simulink model "tb_sim_monitors"  (R2026b)
undefined symbols (not defined in the file or in its folder): Ts
settings Model: Creator=aomar  LastModifiedBy=aomar

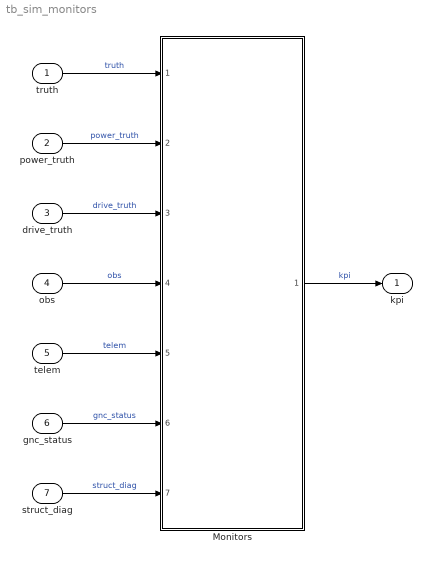
== system tb_sim_monitors ==
  truth : Inport  OutDataTypeStr=Bus: Bus_TruthState  SampleTime=Ts.base  BusOutputAsStruct=on
  power_truth : Inport  Port=2  OutDataTypeStr=Bus: Bus_PowerTruth  SampleTime=Ts.hk  BusOutputAsStruct=on
  drive_truth : Inport  Port=3  OutDataTypeStr=Bus: Bus_DriveTruth  SampleTime=Ts.base  BusOutputAsStruct=on
  obs : Inport  Port=4  OutDataTypeStr=Bus: Bus_ObstaclesDyn  SampleTime=Ts.ctrl  BusOutputAsStruct=on
  telem : Inport  Port=5  OutDataTypeStr=Bus: Bus_FwTelemetry  SampleTime=Ts.ctrl  BusOutputAsStruct=on
  gnc_status : Inport  Port=6  OutDataTypeStr=Bus: Bus_GncStatus  SampleTime=Ts.gnc_status  BusOutputAsStruct=on
  struct_diag : Inport  Port=7  OutDataTypeStr=Bus: Bus_StructureDiag  SampleTime=Ts.ctrl  BusOutputAsStruct=on
  Monitors : Subsystem  ReferencedSubsystem=Sim_Monitors
  kpi : Outport  OutDataTypeStr=Bus: Bus_SimKPI
  wires:
  truth/1 -> Monitors/1  "truth"
  power_truth/1 -> Monitors/2  "power_truth"
  drive_truth/1 -> Monitors/3  "drive_truth"
  obs/1 -> Monitors/4  "obs"
  telem/1 -> Monitors/5  "telem"
  gnc_status/1 -> Monitors/6  "gnc_status"
  struct_diag/1 -> Monitors/7  "struct_diag"
  Monitors/1 -> kpi/1  "kpi"
